simulink model "Template_v5_0_0_2026a_Original"  (R2026a)
settings: Solver=ode4  StopTime=tsim  FixedStep=baseRate  RelTol=1e-6  AbsTol=1e-6
undefined symbols (not defined in the file or in its folder): baseRate, dataRate, DiscIntNeverNeededParam, F_thrusters_BLACK, F_thrusters_BLUE, F_thrusters_RED, home_states_BLACK, home_states_BLUE, home_states_RED, IBLACK, IBLUE, init_states_BLACK, init_states_BLUE, init_states_RED, IRED, K_BLACK, K_BLUE, K_RED, labConsoleIP, mBLACK, mBLUE, mRED, Phase0_End, Phase1_End, Phase2_End, Phase3_End, Phase3_SubPhase1_End, Phase3_SubPhase2_End, Phase3_SubPhase3_End, Phase3_SubPhase4_End, Phase4_End, Phase5_End, platformSelection, PWMFreq, serverRate, simMode, tableDamping_BLACK, tableDamping_BLUE, tableDamping_RED, tableSlope, thrust_decay_BLACK, thrust_decay_BLUE, thrust_decay_RED, thruster_dist2CG_BLACK, thruster_dist2CG_BLUE, thruster_dist2CG_RED, xLength, yLength
libraries: simulink x18, dspinverses x3, nvidiaCommlib x1
(part 3 of 7)

== system Template_v5_0_0_2026a_Original/4 - Control/Disable Control (ARM) ==
  Action Port : ActionPort  ActionPortLabel=else
  Constant7 : Constant  Value=0
  Data Store Write12 : DataStoreWrite  DataStoreName=ARM_Control_Mode  IndexOptions=Index vector (dialog)  Indices=1  OutputSizes=1
  Mux : Mux  Inputs=3
  Zero : Constant  Value=0  OutDataTypeStr=Inherit: Inherit via back propagation
  Out1 : Outport
  wires:
  Mux/1 -> Out1/1
  Zero/1 -> Mux/3, Mux/1, Mux/2
  Constant7/1 -> Data Store Write12/1

== system Template_v5_0_0_2026a_Original/4 - Control/Disable Thrusters (BLACK) ==
  Action Port : ActionPort  ActionPortLabel=else
  Mux : Mux  Inputs=3
  Zero : Constant  Value=0  OutDataTypeStr=Inherit: Inherit via back propagation
  Out1 : Outport
  wires:
  Zero/1 -> Mux/3, Mux/1, Mux/2
  Mux/1 -> Out1/1

== system Template_v5_0_0_2026a_Original/4 - Control/Disable Thrusters (BLUE) ==
  Action Port : ActionPort  ActionPortLabel=else
  Mux : Mux  Inputs=3
  Zero : Constant  Value=0  OutDataTypeStr=Inherit: Inherit via back propagation
  Out1 : Outport
  wires:
  Zero/1 -> Mux/3, Mux/1, Mux/2
  Mux/1 -> Out1/1

== system Template_v5_0_0_2026a_Original/4 - Control/Disable Thrusters (RED) ==
  Action Port : ActionPort  ActionPortLabel=else
  Mux : Mux  Inputs=3
  Zero : Constant  Value=0  OutDataTypeStr=Inherit: Inherit via back propagation
  u : Outport
  wires:
  Zero/1 -> Mux/3, Mux/1, Mux/2
  Mux/1 -> u/1

== system Template_v5_0_0_2026a_Original/Check Connection/Change BLACK Behavior ==
  Action Port : ActionPort  ActionPortLabel=if(u1 == 2 & u2 == 0)
  Constant1 : Constant  OutDataTypeStr=int32
  UDP Send : MATLAB Function  TreatAsAtomicUnit=on
  wires:
  Constant1/1 -> UDP Send/1(data)

== system Template_v5_0_0_2026a_Original/Check Connection/Change BLUE Behavior ==
  Action Port : ActionPort  ActionPortLabel=if(u1 == 3 & u2 == 0)
  Constant1 : Constant  OutDataTypeStr=int32
  UDP Send : MATLAB Function  TreatAsAtomicUnit=on
  wires:
  Constant1/1 -> UDP Send/1(data)

== system Template_v5_0_0_2026a_Original/Check Connection/Change RED Behavior ==
  Action Port : ActionPort  ActionPortLabel=if(u1 == 1 & u2 == 0)
  Constant1 : Constant  OutDataTypeStr=int32
  UDP Send : MATLAB Function  TreatAsAtomicUnit=on
  wires:
  Constant1/1 -> UDP Send/1(data)

== system Template_v5_0_0_2026a_Original/Data Logger Subsystem/Data Logger ==
  Data : Inport
  MATLAB Function : MATLAB Function  TreatAsAtomicUnit=on
  MATLAB System : MATLABSystem  System=spot.hardware.CustomDataLogger
      mask Type: spot.hardware.CustomDataLogger
  wires:
  MATLAB Function/1(inputSize) -> MATLAB System/2
  Data/1 -> MATLAB System/1, MATLAB Function/1(Input)

== system Template_v5_0_0_2026a_Original/Live Data Streams/Live Stream 1 ==
  u : Inport
  Stream : MATLAB Function  TreatAsAtomicUnit=on
  Univ_Time : DataStoreRead  DataStoreName=Univ_Time  IndexOptions=Index vector (dialog)  Indices=1  OutputSizes=1
  WhoAmI : DataStoreRead  DataStoreName=WhoAmI  IndexOptions=Index vector (dialog)  Indices=1  OutputSizes=1
  isSim : DataStoreRead  DataStoreName=isSim  IndexOptions=Index vector (dialog)  Indices=1  OutputSizes=1
  wires:
  u/1 -> Stream/1(u)
  Univ_Time/1 -> Stream/2(t)
  WhoAmI/1 -> Stream/3(whoAmI)
  isSim/1 -> Stream/4(isSim)

== system Template_v5_0_0_2026a_Original/Live Data Streams/Live Stream 2 ==
  u : Inport
  Stream : MATLAB Function  TreatAsAtomicUnit=on
  Univ_Time : DataStoreRead  DataStoreName=Univ_Time  IndexOptions=Index vector (dialog)  Indices=1  OutputSizes=1
  WhoAmI : DataStoreRead  DataStoreName=WhoAmI  IndexOptions=Index vector (dialog)  Indices=1  OutputSizes=1
  isSim : DataStoreRead  DataStoreName=isSim  IndexOptions=Index vector (dialog)  Indices=1  OutputSizes=1
  wires:
  u/1 -> Stream/1(u)
  Univ_Time/1 -> Stream/2(t)
  WhoAmI/1 -> Stream/3(whoAmI)
  isSim/1 -> Stream/4(isSim)

== system Template_v5_0_0_2026a_Original/Live Data Streams/Live Stream 3 ==
  u : Inport
  Stream : MATLAB Function  TreatAsAtomicUnit=on
  Univ_Time : DataStoreRead  DataStoreName=Univ_Time  IndexOptions=Index vector (dialog)  Indices=1  OutputSizes=1
  WhoAmI : DataStoreRead  DataStoreName=WhoAmI  IndexOptions=Index vector (dialog)  Indices=1  OutputSizes=1
  isSim : DataStoreRead  DataStoreName=isSim  IndexOptions=Index vector (dialog)  Indices=1  OutputSizes=1
  wires:
  u/1 -> Stream/1(u)
  Univ_Time/1 -> Stream/2(t)
  WhoAmI/1 -> Stream/3(whoAmI)
  isSim/1 -> Stream/4(isSim)

== system Template_v5_0_0_2026a_Original/Live Data Streams/Live Stream 4 ==
  u : Inport
  Stream : MATLAB Function  TreatAsAtomicUnit=on
  Univ_Time : DataStoreRead  DataStoreName=Univ_Time  IndexOptions=Index vector (dialog)  Indices=1  OutputSizes=1
  WhoAmI : DataStoreRead  DataStoreName=WhoAmI  IndexOptions=Index vector (dialog)  Indices=1  OutputSizes=1
  isSim : DataStoreRead  DataStoreName=isSim  IndexOptions=Index vector (dialog)  Indices=1  OutputSizes=1
  wires:
  u/1 -> Stream/1(u)
  Univ_Time/1 -> Stream/2(t)
  WhoAmI/1 -> Stream/3(whoAmI)
  isSim/1 -> Stream/4(isSim)

== system Template_v5_0_0_2026a_Original/PhaseSpace Camera Code/Initialize Universal Time (Simulation) ==
  Action Port : ActionPort  ActionPortLabel=elseif(u1 == 1)
  Set Universal Time (If this is a simulation) : Clock
  Universal_Time : DataStoreWrite  DataStoreName=Univ_Time  IndexOptions=Index vector (dialog)  Indices=1  OutputSizes=1
  wires:
  Set Universal Time (If this is a simulation)/1 -> Universal_Time/1

== system Template_v5_0_0_2026a_Original/PhaseSpace Camera Code/Use Hardware to Obtain States ==
  Action Port : ActionPort  ActionPortLabel=if(u1 == 0)
  Demux : Demux  Outputs=[4,3,3,9]
  Demux1 : Demux  Outputs=[3,3,3]
  Receive and Process Phasespace Data : Subsystem
  Store BLACK Data : Subsystem
  Store BLUE Data : Subsystem
  Store RED Data : Subsystem
  wires:
  Receive and Process Phasespace Data/1(PhaseSpace Data) -> Demux/1
  Demux/1 -> Store RED Data/1(RED Data)
  Demux/2 -> Store BLACK Data/1(BLACK Data)
  Demux/3 -> Store BLUE Data/1(BLUE Data)
  Demux/4 -> Demux1/1
  Demux1/1 -> Store RED Data/2(RED Velocities)
  Demux1/2 -> Store BLACK Data/2(BLACK Velocities)
  Demux1/3 -> Store BLUE Data/2(BLUE Velocities)
  Receive and Process Phasespace Data/2(PhaseSpace Clock) -> Store RED Data/3(PS Clock), Store BLACK Data/3(PS Clock), Store BLUE Data/3(PS Clock)

== system Template_v5_0_0_2026a_Original/Platform Identification/Subsystem ==
  Action Port : ActionPort  ActionPortLabel=if(u1 == 0)
  Data Store Write : DataStoreWrite  DataStoreName=WhoAmI  IndexOptions=Index vector (dialog)  Indices=1  OutputSizes=1
  WhoAmI : MATLABSystem  System=spot.hardware.IdentifyPlatform  SampleTime=baseRate
      mask Type: spot.hardware.IdentifyPlatform
  wires:
  WhoAmI/1 -> Data Store Write/1

== system Template_v5_0_0_2026a_Original/Receive Data from Orin/Subsystem ==
  Action Port : ActionPort  ActionPortLabel=if(u1 == 0)
  Cast To Double{,1..3} (4 alike) : DataTypeConversion  OutDataTypeStr=double  SaturateOnIntegerOverflow=off  RndMeth=Floor
  Data Store Write : DataStoreWrite  DataStoreName=VIS_Measured_States  IndexOptions=Index vector (dialog)  Indices=1  OutputSizes=1
  Data Store Write1 : DataStoreWrite  DataStoreName=VIS_Confidence  IndexOptions=Index vector (dialog)  Indices=1  OutputSizes=1
  Demux : Demux
  Mux : Mux  Inputs=3
  Terminator : Terminator
  Terminator1 : Terminator
  UDP Receive : MATLAB Function  TreatAsAtomicUnit=on
  wires:
  Demux/1 -> Cast To Double/1
  Demux/2 -> Cast To Double1/1
  Demux/3 -> Cast To Double2/1
  Demux/4 -> Cast To Double3/1
  Cast To Double/1 -> Mux/1
  Cast To Double1/1 -> Mux/2
  Cast To Double2/1 -> Mux/3
  Mux/1 -> Data Store Write/1
  Cast To Double3/1 -> Data Store Write1/1
  UDP Receive/1(data) -> Demux/1
  UDP Receive/2(newPackets) -> Terminator/1
  UDP Receive/3(age) -> Terminator1/1

== system Template_v5_0_0_2026a_Original/Robotic Arm Code/Change ARM Behavior ==
  note: Reads the encoders here (priority 21, before the controllers); sends the PWM input (ARM_Controls, from Robotic Arm Code) at the end of the step. See help spot.hardware.ArmPWM.
  PWM : Inport
  Action Port : ActionPort  ActionPortLabel=if(u1 == 1 & u2 == 0)
  Data Store Write : DataStoreWrite  DataStoreName=ARM_Measured_States  IndexOptions=Index vector (dialog)  Indices=1  OutputSizes=1
  Data Store Write1 : DataStoreWrite  DataStoreName=ARM_Measured_PWM  IndexOptions=Index vector (dialog)  Indices=1  OutputSizes=1
  Data Store Write2 : DataStoreWrite  DataStoreName=ARM_Servo_Status  IndexOptions=Index vector (dialog)  Indices=1  OutputSizes=1
  Dynamixel Arm (PWM) : MATLABSystem  System=spot.hardware.ArmPWM  Port=/dev/ttyUSB0  PWMLimit=885  ZeroReturnDelay=off  MinPosition=1024  MaxPosition=3072
      mask Type: spot.hardware.ArmPWM
  Mux : Mux  Inputs=2
  wires:
  Dynamixel Arm (PWM)/1 -> Mux/1
  Dynamixel Arm (PWM)/2 -> Mux/2
  Mux/1 -> Data Store Write/1
  Dynamixel Arm (PWM)/3 -> Data Store Write1/1
  Dynamixel Arm (PWM)/4 -> Data Store Write2/1
  PWM/1 -> Dynamixel Arm (PWM)/1

== system Template_v5_0_0_2026a_Original/Send Data to Orin/Subsystem ==
  Action Port : ActionPort  ActionPortLabel=if(u1 == 0)
  BLACK States : DataStoreRead  DataStoreName=BLACK_Measured_States  IndexOptions=Index vector (dialog)  Indices=1  OutputSizes=1
  BLUE States : DataStoreRead  DataStoreName=BLUE_Measured_States  IndexOptions=Index vector (dialog)  Indices=1  OutputSizes=1
  Mux : Mux
  RED States : DataStoreRead  DataStoreName=RED_Measured_States  IndexOptions=Index vector (dialog)  Indices=1  OutputSizes=1
  Time : DataStoreRead  DataStoreName=Univ_Time  IndexOptions=Index vector (dialog)  Indices=1  OutputSizes=1
  UDP Send : MATLAB Function  TreatAsAtomicUnit=on
  wires:
  Time/1 -> Mux/1
  RED States/1 -> Mux/2
  BLACK States/1 -> Mux/3
  BLUE States/1 -> Mux/4
  Mux/1 -> UDP Send/1(data)

== system Template_v5_0_0_2026a_Original/Simulate Plant Dynamics/BLACK Dynamics ==
  Add Noise : RandomNumber  Variance=1e-9  SampleTime=baseRate
  Calculated & Store Measured States : Subsystem
  Calculated & Store True States : Subsystem
  Data @ Measurement Rate : Subsystem
  Dynamics Model for BLACK : Subsystem  SystemSampleTime=serverRate
      settings: PortSchema="{\"entries\":[{\"content\":{\"sides\":[{\"content\":{\"connectorIds\":[\"In1\"]},\"type\":\"ConnectorPlacement.EquallySpacedRectSide\",\"uuid\":\"9df3cfb7-f920-4c45-b004-2d63eab5f007\"},{\"content\":{\"side\":\"RIGHT\"},\"type\":\"ConnectorPlacement.EquallySpacedRectSide\",\"uuid\":\"24f4b70f-864f-4cab-bc2b-b450467a01b3\"},{\"content\":{\"connectorIds\":[\"Out1\"],\"side\":\"TOP\"},\"type\":\"ConnectorPlacement.EquallySpacedRectSide\",\"uuid\":\"64c0236c-f70a-4099-950e-ee3e8643e7f2\"}]},\"type\":\"ConnectorPlacement.EquallySpacedConnector\",\"uuid\":\"dd7c693a-185b-4c5f-873e-b9df56bea395\"}],\"packageUris\":[\"http://schema.mathworks.com/mf0/Connector/R2020b\"],\"version\":\"1.0\"}"
  Saturated Control Commands for BLACK : DataStoreRead  DataStoreName=BLACK_Saturated_Controls  IndexOptions=Index vector (dialog)  Indices=1  OutputSizes=1
  Sum : Sum  Inputs=++|
  wires:
  Dynamics Model for BLACK/1(states) -> Sum/2, Calculated & Store True States/1(y)
  Data @ Measurement Rate/2(Time Step) -> Calculated & Store Measured States/2(dt)
  Saturated Control Commands for BLACK/1 -> Dynamics Model for BLACK/1(control_inputs)
  Data @ Measurement Rate/1(Data Held) -> Calculated & Store Measured States/1(y)
  Sum/1 -> Data @ Measurement Rate/1(Data Input)
  Add Noise/1 -> Sum/1

== system Template_v5_0_0_2026a_Original/Simulate Plant Dynamics/BLUE Dynamics ==
  Add Noise : RandomNumber  Variance=1e-9  SampleTime=baseRate
  BLUE  Dynamics Model : Subsystem  SystemSampleTime=serverRate
      settings: PortSchema="{\"entries\":[{\"content\":{\"sides\":[{\"content\":{\"connectorIds\":[\"In1\"]},\"type\":\"ConnectorPlacement.EquallySpacedRectSide\",\"uuid\":\"9df3cfb7-f920-4c45-b004-2d63eab5f007\"},{\"content\":{\"side\":\"RIGHT\"},\"type\":\"ConnectorPlacement.EquallySpacedRectSide\",\"uuid\":\"24f4b70f-864f-4cab-bc2b-b450467a01b3\"},{\"content\":{\"connectorIds\":[\"Out1\"],\"side\":\"TOP\"},\"type\":\"ConnectorPlacement.EquallySpacedRectSide\",\"uuid\":\"64c0236c-f70a-4099-950e-ee3e8643e7f2\"}]},\"type\":\"ConnectorPlacement.EquallySpacedConnector\",\"uuid\":\"dd7c693a-185b-4c5f-873e-b9df56bea395\"}],\"packageUris\":[\"http://schema.mathworks.com/mf0/Connector/R2020b\"],\"version\":\"1.0\"}"
  Calculated & Store Measured States : Subsystem
  Calculated & Store True States : Subsystem
  Data @ Measurement Rate : Subsystem
  Saturated Control Commands for BLUE : DataStoreRead  DataStoreName=BLUE_Saturated_Controls  IndexOptions=Index vector (dialog)  Indices=1  OutputSizes=1
  Sum1 : Sum  Inputs=++|
  wires:
  Saturated Control Commands for BLUE/1 -> BLUE  Dynamics Model/1(control_inputs)
  Data @ Measurement Rate/2(Time Step) -> Calculated & Store Measured States/2(dt)
  Add Noise/1 -> Sum1/1
  BLUE  Dynamics Model/1(states) -> Sum1/2, Calculated & Store True States/1(y)
  Sum1/1 -> Data @ Measurement Rate/1(Data Input)
  Data @ Measurement Rate/1(Data Held) -> Calculated & Store Measured States/1(y)

== system Template_v5_0_0_2026a_Original/Simulate Plant Dynamics/RED and ARM Dynamics ==
  Constant : Constant  Value=platformSelection
  If : If  IfExpression=u1 == 4 | u1 == 5 | u1 == 10 | u1 == 11
  RED + ARM : Subsystem  TreatAsAtomicUnit=on
  RED Only : Subsystem  TreatAsAtomicUnit=on
  wires:
  If/1 -> RED + ARM/Action
  Constant/1 -> If/1
  If/2 -> RED Only/Action

== system Template_v5_0_0_2026a_Original/Thruster & Float Control Code/Change BLACK Behavior ==
  note: Calculate the percentage of time each thruster must be on, and send to the PWM blocks.
  note: Using the attitude, rotate the forces into the body frame.
  note: Calculate which thrusters must be turned on and for how long.
  Action Port : ActionPort  ActionPortLabel=if(u1 == 2 | u2 == 1)
  BLACK Controls : DataStoreRead  DataStoreName=BLACK_Controls  IndexOptions=Index vector (dialog)  Indices=1  OutputSizes=1
  BLACK States : DataStoreRead  DataStoreName=BLACK_Measured_States  IndexOptions=Index vector (dialog)  Indices=1  OutputSizes=1
  Calculate Duty Cycle : Subsystem
  Data Store Write2 : DataStoreWrite  DataStoreName=BLACK_Saturated_Controls  IndexOptions=Index vector (dialog)  Indices=1  OutputSizes=1
  Demux1 : Demux  Outputs=[2,1]
  Demux2 : Demux  Outputs=[2,1,6]
  Mux : Mux  Inputs=2
  Rotate Forces to Body : Subsystem
  Terminator : Terminator
  Terminator1 : Terminator
  BLACK DC : Outport  VectorParamsAs1DForOutWhenUnconnected=off
  wires:
  Calculate Duty Cycle/2(Saturated Forces Moments) -> Data Store Write2/1
  Rotate Forces to Body/1(F_b) -> Mux/1
  Demux1/2 -> Mux/2
  Calculate Duty Cycle/1(Duty Cycle) -> BLACK DC/1
  Mux/1 -> Calculate Duty Cycle/1("[Fx_b; Fy_b; Tz]")
  BLACK Controls/1 -> Demux1/1
  Demux1/1 -> Rotate Forces to Body/1("F_I ")
  BLACK States/1 -> Demux2/1
  Demux2/1 -> Terminator/1
  Demux2/3 -> Terminator1/1
  Demux2/2 -> Calculate Duty Cycle/2(Measured Attitude), Rotate Forces to Body/2(Rz)

== system Template_v5_0_0_2026a_Original/Thruster & Float Control Code/Change BLUE Behavior ==
  note: Calculate the percentage of time each thruster must be on, and send to the PWM blocks.
  note: Using the attitude, rotate the forces into the body frame.
  note: Calculate which thrusters must be turned on and for how long.
  Action Port : ActionPort  ActionPortLabel=if(u1 == 3 | u2 == 1)
  Calculate Duty Cycle : Subsystem
  Data Store Read : DataStoreRead  DataStoreName=BLUE_Controls  IndexOptions=Index vector (dialog)  Indices=1  OutputSizes=1
  Data Store Read1 : DataStoreRead  DataStoreName=BLUE_Measured_States  IndexOptions=Index vector (dialog)  Indices=1  OutputSizes=1
  Data Store Write3 : DataStoreWrite  DataStoreName=BLUE_Saturated_Controls  IndexOptions=Index vector (dialog)  Indices=1  OutputSizes=1
  Demux : Demux  Outputs=[2,1]
  Demux1 : Demux  Outputs=[2,1,6]
  Mux1 : Mux  Inputs=2
  Rotate Forces to Body : Subsystem
  Terminator : Terminator
  Terminator1 : Terminator
  BLUE DC : Outport  VectorParamsAs1DForOutWhenUnconnected=off
  wires:
  Calculate Duty Cycle/1(Duty Cycle) -> BLUE DC/1
  Rotate Forces to Body/1(F_b) -> Mux1/1
  Demux/2 -> Mux1/2
  Mux1/1 -> Calculate Duty Cycle/1("[Fx_b; Fy_b; Tz]")
  Calculate Duty Cycle/2(Saturated Forces Moments) -> Data Store Write3/1
  Data Store Read/1 -> Demux/1
  Demux/1 -> Rotate Forces to Body/1("F_I ")
  Data Store Read1/1 -> Demux1/1
  Demux1/2 -> Calculate Duty Cycle/2(Measured Attitude), Rotate Forces to Body/2(Rz)
  Demux1/1 -> Terminator/1
  Demux1/3 -> Terminator1/1

== system Template_v5_0_0_2026a_Original/Thruster & Float Control Code/Change RED Behavior ==
  note: Calculate which thrusters must be turned on and for how long.
  note: Calculate the percentage of time each thruster must be on, and send to the PWM blocks.
  note: Using the attitude, rotate the forces into the body frame.
  Action Port : ActionPort  ActionPortLabel=if(u1 == 1 | u2 == 1)
  Calculate Duty Cycle : Subsystem
  Data Store Read : DataStoreRead  DataStoreName=RED_Controls  IndexOptions=Index vector (dialog)  Indices=1  OutputSizes=1
  Data Store Read1 : DataStoreRead  DataStoreName=RED_Measured_States  IndexOptions=Index vector (dialog)  Indices=1  OutputSizes=1
  Data Store Write1 : DataStoreWrite  DataStoreName=RED_Saturated_Controls  IndexOptions=Index vector (dialog)  Indices=1  OutputSizes=1
  Demux : Demux  Outputs=[2,1]
  Demux1 : Demux  Outputs=[2,1,6]
  Mux1 : Mux  Inputs=2
  Rotate Forces to Body : Subsystem
  Terminator : Terminator
  Terminator1 : Terminator
  RED DC : Outport  VectorParamsAs1DForOutWhenUnconnected=off
  wires:
  Demux/1 -> Rotate Forces to Body/1("F_I ")
  Mux1/1 -> Calculate Duty Cycle/1("[Fx_b; Fy_b; Tz]")
  Demux/2 -> Mux1/2
  Demux1/2 -> Calculate Duty Cycle/2(Measured Attitude), Rotate Forces to Body/2(Rz)
  Rotate Forces to Body/1(F_b) -> Mux1/1
  Data Store Read/1 -> Demux/1
  Demux1/1 -> Terminator/1
  Demux1/3 -> Terminator1/1
  Data Store Read1/1 -> Demux1/1
  Calculate Duty Cycle/2(Saturated Forces Moments) -> Data Store Write1/1
  Calculate Duty Cycle/1(Duty Cycle) -> RED DC/1

== system Template_v5_0_0_2026a_Original/1 - Experiment Logic/Phase #2: Initial Position/Desired Joint Angles RED ==
  Constant1 : Constant  Value=pi/2
  Constant2 : Constant  Value=0
  Constant3 : Constant  Value=pi/2
  Mux : Mux  Inputs=3
  Target Array : Outport
  wires:
  Mux/1 -> Target Array/1
  Constant3/1 -> Mux/1
  Constant1/1 -> Mux/2
  Constant2/1 -> Mux/3

== system Template_v5_0_0_2026a_Original/1 - Experiment Logic/Phase #2: Initial Position/Desired Position BLACK ==
  Desired States (BLACK) : Constant  Value=init_states_BLACK  SampleTime=-1
  Target Array : Outport
  wires:
  Desired States (BLACK)/1 -> Target Array/1

== system Template_v5_0_0_2026a_Original/1 - Experiment Logic/Phase #2: Initial Position/Desired Position BLUE ==
  Desired States (BLUE) : Constant  Value=init_states_BLUE  SampleTime=-1
  Target Array : Outport
  wires:
  Desired States (BLUE)/1 -> Target Array/1

== system Template_v5_0_0_2026a_Original/1 - Experiment Logic/Phase #2: Initial Position/Desired Position RED ==
  Constant2 : Constant  Value=init_states_RED
  Target Array : Outport
  wires:
  Constant2/1 -> Target Array/1

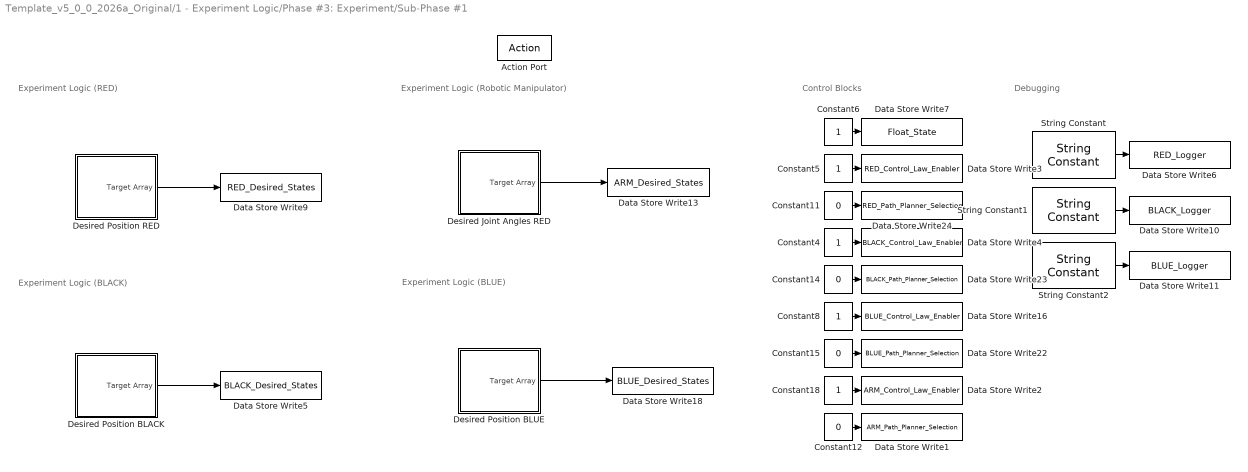
== system Template_v5_0_0_2026a_Original/1 - Experiment Logic/Phase #3: Experiment/Sub-Phase #1 ==
  note: Experiment Logic (BLUE)
  note: Experiment Logic (Robotic Manipulator)
  note: Experiment Logic (RED)
  note: Experiment Logic (BLACK)
  note: Control Blocks
  note: Debugging
  Action Port : ActionPort  ActionPortLabel=if(u1 < u2)
  Constant{11..12,14..15} (4 alike) : Constant  Value=0
  Constant{4..6,8,18} (5 alike) : Constant
  Data Store Write1 : DataStoreWrite  DataStoreName=ARM_Path_Planner_Selection  IndexOptions=Index vector (dialog)  Indices=1  OutputSizes=1
  Data Store Write10 : DataStoreWrite  DataStoreName=BLACK_Logger  IndexOptions=Index vector (dialog)  Indices=1  OutputSizes=1
  Data Store Write11 : DataStoreWrite  DataStoreName=BLUE_Logger  IndexOptions=Index vector (dialog)  Indices=1  OutputSizes=1
  Data Store Write13 : DataStoreWrite  DataStoreName=ARM_Desired_States  IndexOptions=Index vector (dialog)  Indices=1  OutputSizes=1
  Data Store Write16 : DataStoreWrite  DataStoreName=BLUE_Control_Law_Enabler  IndexOptions=Index vector (dialog)  Indices=1  OutputSizes=1
  Data Store Write18 : DataStoreWrite  DataStoreName=BLUE_Desired_States  IndexOptions=Index vector (dialog)  Indices=1  OutputSizes=1
  Data Store Write2 : DataStoreWrite  DataStoreName=ARM_Control_Law_Enabler  IndexOptions=Index vector (dialog)  Indices=1  OutputSizes=1
  Data Store Write22 : DataStoreWrite  DataStoreName=BLUE_Path_Planner_Selection  IndexOptions=Index vector (dialog)  Indices=1  OutputSizes=1
  Data Store Write23 : DataStoreWrite  DataStoreName=BLACK_Path_Planner_Selection  IndexOptions=Index vector (dialog)  Indices=1  OutputSizes=1
  Data Store Write24 : DataStoreWrite  DataStoreName=RED_Path_Planner_Selection  IndexOptions=Index vector (dialog)  Indices=1  OutputSizes=1
  Data Store Write3 : DataStoreWrite  DataStoreName=RED_Control_Law_Enabler  IndexOptions=Index vector (dialog)  Indices=1  OutputSizes=1
  Data Store Write4 : DataStoreWrite  DataStoreName=BLACK_Control_Law_Enabler  IndexOptions=Index vector (dialog)  Indices=1  OutputSizes=1
  Data Store Write5 : DataStoreWrite  DataStoreName=BLACK_Desired_States  IndexOptions=Index vector (dialog)  Indices=1  OutputSizes=1
  Data Store Write6 : DataStoreWrite  DataStoreName=RED_Logger  IndexOptions=Index vector (dialog)  Indices=1  OutputSizes=1
  Data Store Write7 : DataStoreWrite  DataStoreName=Float_State  IndexOptions=Index vector (dialog)  Indices=1  OutputSizes=1
  Data Store Write9 : DataStoreWrite  DataStoreName=RED_Desired_States  IndexOptions=Index vector (dialog)  Indices=1  OutputSizes=1
  Desired Joint Angles RED : Subsystem
  Desired Position BLACK : Subsystem
  Desired Position BLUE : Subsystem
  Desired Position RED : Subsystem
  String Constant : StringConstant  String="\"Chaser: Running Phase 3 Sub-Phase 1\""
  String Constant1 : StringConstant  String="\"Target: Running Phase 3 Sub-Phase 1\""
  String Constant2 : StringConstant  String="\"Obstacle: Running Phase 3 Sub-Phase 1\""
  wires:
  Desired Position BLUE/1(Target Array) -> Data Store Write18/1
  Desired Position RED/1(Target Array) -> Data Store Write9/1
  Desired Joint Angles RED/1(Target Array) -> Data Store Write13/1
  Constant12/1 -> Data Store Write1/1
  Constant18/1 -> Data Store Write2/1
  Constant6/1 -> Data Store Write7/1
  Constant15/1 -> Data Store Write22/1
  Constant14/1 -> Data Store Write23/1
  Constant5/1 -> Data Store Write3/1
  Constant11/1 -> Data Store Write24/1
  Constant8/1 -> Data Store Write16/1
  Constant4/1 -> Data Store Write4/1
  String Constant2/1 -> Data Store Write11/1
  String Constant1/1 -> Data Store Write10/1
  String Constant/1 -> Data Store Write6/1
  Desired Position BLACK/1(Target Array) -> Data Store Write5/1

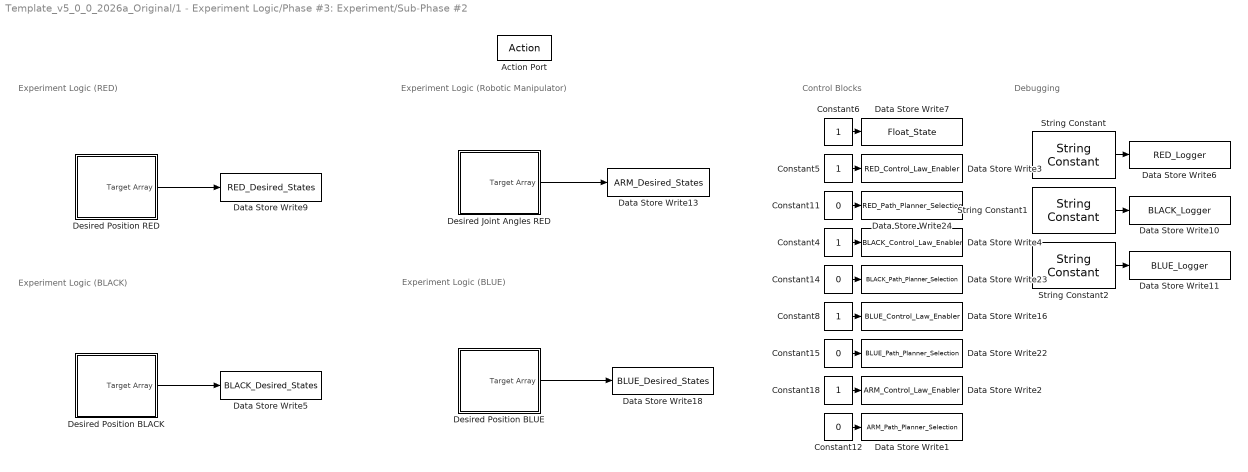
== system Template_v5_0_0_2026a_Original/1 - Experiment Logic/Phase #3: Experiment/Sub-Phase #2 ==
  note: Experiment Logic (BLUE)
  note: Experiment Logic (Robotic Manipulator)
  note: Experiment Logic (RED)
  note: Experiment Logic (BLACK)
  note: Control Blocks
  note: Debugging
  Action Port : ActionPort  ActionPortLabel=elseif((u1 < u3 & u1 >= u2))
  Constant{11..12,14..15} (4 alike) : Constant  Value=0
  Constant{4..6,8,18} (5 alike) : Constant
  Data Store Write1 : DataStoreWrite  DataStoreName=ARM_Path_Planner_Selection  IndexOptions=Index vector (dialog)  Indices=1  OutputSizes=1
  Data Store Write10 : DataStoreWrite  DataStoreName=BLACK_Logger  IndexOptions=Index vector (dialog)  Indices=1  OutputSizes=1
  Data Store Write11 : DataStoreWrite  DataStoreName=BLUE_Logger  IndexOptions=Index vector (dialog)  Indices=1  OutputSizes=1
  Data Store Write13 : DataStoreWrite  DataStoreName=ARM_Desired_States  IndexOptions=Index vector (dialog)  Indices=1  OutputSizes=1
  Data Store Write16 : DataStoreWrite  DataStoreName=BLUE_Control_Law_Enabler  IndexOptions=Index vector (dialog)  Indices=1  OutputSizes=1
  Data Store Write18 : DataStoreWrite  DataStoreName=BLUE_Desired_States  IndexOptions=Index vector (dialog)  Indices=1  OutputSizes=1
  Data Store Write2 : DataStoreWrite  DataStoreName=ARM_Control_Law_Enabler  IndexOptions=Index vector (dialog)  Indices=1  OutputSizes=1
  Data Store Write22 : DataStoreWrite  DataStoreName=BLUE_Path_Planner_Selection  IndexOptions=Index vector (dialog)  Indices=1  OutputSizes=1
  Data Store Write23 : DataStoreWrite  DataStoreName=BLACK_Path_Planner_Selection  IndexOptions=Index vector (dialog)  Indices=1  OutputSizes=1
  Data Store Write24 : DataStoreWrite  DataStoreName=RED_Path_Planner_Selection  IndexOptions=Index vector (dialog)  Indices=1  OutputSizes=1
  Data Store Write3 : DataStoreWrite  DataStoreName=RED_Control_Law_Enabler  IndexOptions=Index vector (dialog)  Indices=1  OutputSizes=1
  Data Store Write4 : DataStoreWrite  DataStoreName=BLACK_Control_Law_Enabler  IndexOptions=Index vector (dialog)  Indices=1  OutputSizes=1
  Data Store Write5 : DataStoreWrite  DataStoreName=BLACK_Desired_States  IndexOptions=Index vector (dialog)  Indices=1  OutputSizes=1
  Data Store Write6 : DataStoreWrite  DataStoreName=RED_Logger  IndexOptions=Index vector (dialog)  Indices=1  OutputSizes=1
  Data Store Write7 : DataStoreWrite  DataStoreName=Float_State  IndexOptions=Index vector (dialog)  Indices=1  OutputSizes=1
  Data Store Write9 : DataStoreWrite  DataStoreName=RED_Desired_States  IndexOptions=Index vector (dialog)  Indices=1  OutputSizes=1
  Desired Joint Angles RED : Subsystem
  Desired Position BLACK : Subsystem
  Desired Position BLUE : Subsystem
  Desired Position RED : Subsystem
  String Constant : StringConstant  String="\"Chaser: Running Phase 3 Sub-Phase 2\""
  String Constant1 : StringConstant  String="\"Target: Running Phase 3 Sub-Phase 2\""
  String Constant2 : StringConstant  String="\"Obstacle: Running Phase 3 Sub-Phase 2\""
  wires:
  Desired Position BLUE/1(Target Array) -> Data Store Write18/1
  Desired Position RED/1(Target Array) -> Data Store Write9/1
  Desired Joint Angles RED/1(Target Array) -> Data Store Write13/1
  Constant12/1 -> Data Store Write1/1
  Constant18/1 -> Data Store Write2/1
  Constant6/1 -> Data Store Write7/1
  Constant15/1 -> Data Store Write22/1
  Constant14/1 -> Data Store Write23/1
  Constant5/1 -> Data Store Write3/1
  Constant11/1 -> Data Store Write24/1
  Constant8/1 -> Data Store Write16/1
  Constant4/1 -> Data Store Write4/1
  String Constant2/1 -> Data Store Write11/1
  String Constant1/1 -> Data Store Write10/1
  String Constant/1 -> Data Store Write6/1
  Desired Position BLACK/1(Target Array) -> Data Store Write5/1

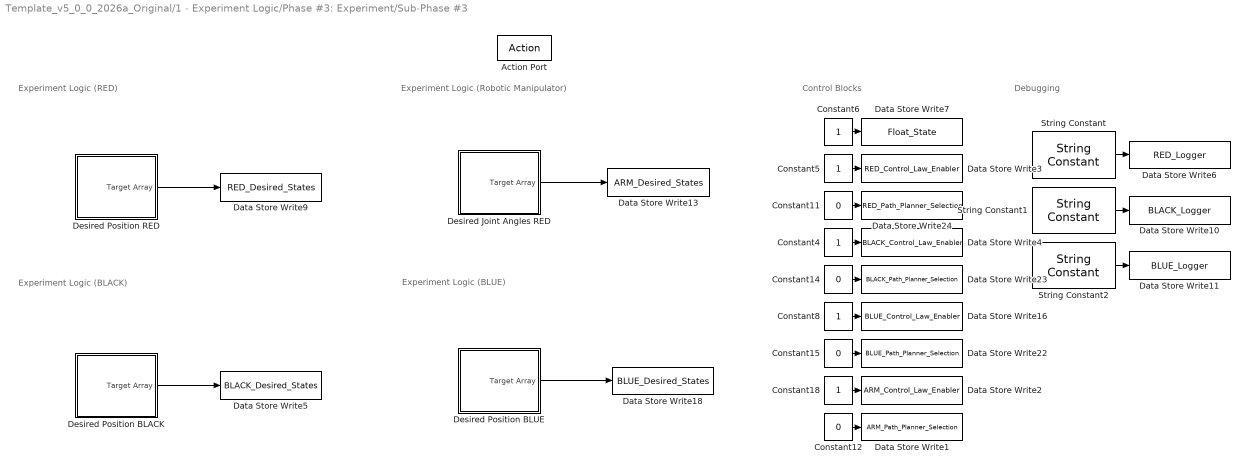
== system Template_v5_0_0_2026a_Original/1 - Experiment Logic/Phase #3: Experiment/Sub-Phase #3 ==
  note: Experiment Logic (BLUE)
  note: Experiment Logic (Robotic Manipulator)
  note: Experiment Logic (RED)
  note: Experiment Logic (BLACK)
  note: Control Blocks
  note: Debugging
  Action Port : ActionPort  ActionPortLabel=elseif((u1 < u4 & u1 >= u3))
  Constant{11..12,14..15} (4 alike) : Constant  Value=0
  Constant{4..6,8,18} (5 alike) : Constant
  Data Store Write1 : DataStoreWrite  DataStoreName=ARM_Path_Planner_Selection  IndexOptions=Index vector (dialog)  Indices=1  OutputSizes=1
  Data Store Write10 : DataStoreWrite  DataStoreName=BLACK_Logger  IndexOptions=Index vector (dialog)  Indices=1  OutputSizes=1
  Data Store Write11 : DataStoreWrite  DataStoreName=BLUE_Logger  IndexOptions=Index vector (dialog)  Indices=1  OutputSizes=1
  Data Store Write13 : DataStoreWrite  DataStoreName=ARM_Desired_States  IndexOptions=Index vector (dialog)  Indices=1  OutputSizes=1
  Data Store Write16 : DataStoreWrite  DataStoreName=BLUE_Control_Law_Enabler  IndexOptions=Index vector (dialog)  Indices=1  OutputSizes=1
  Data Store Write18 : DataStoreWrite  DataStoreName=BLUE_Desired_States  IndexOptions=Index vector (dialog)  Indices=1  OutputSizes=1
  Data Store Write2 : DataStoreWrite  DataStoreName=ARM_Control_Law_Enabler  IndexOptions=Index vector (dialog)  Indices=1  OutputSizes=1
  Data Store Write22 : DataStoreWrite  DataStoreName=BLUE_Path_Planner_Selection  IndexOptions=Index vector (dialog)  Indices=1  OutputSizes=1
  Data Store Write23 : DataStoreWrite  DataStoreName=BLACK_Path_Planner_Selection  IndexOptions=Index vector (dialog)  Indices=1  OutputSizes=1
  Data Store Write24 : DataStoreWrite  DataStoreName=RED_Path_Planner_Selection  IndexOptions=Index vector (dialog)  Indices=1  OutputSizes=1
  Data Store Write3 : DataStoreWrite  DataStoreName=RED_Control_Law_Enabler  IndexOptions=Index vector (dialog)  Indices=1  OutputSizes=1
  Data Store Write4 : DataStoreWrite  DataStoreName=BLACK_Control_Law_Enabler  IndexOptions=Index vector (dialog)  Indices=1  OutputSizes=1
  Data Store Write5 : DataStoreWrite  DataStoreName=BLACK_Desired_States  IndexOptions=Index vector (dialog)  Indices=1  OutputSizes=1
  Data Store Write6 : DataStoreWrite  DataStoreName=RED_Logger  IndexOptions=Index vector (dialog)  Indices=1  OutputSizes=1
  Data Store Write7 : DataStoreWrite  DataStoreName=Float_State  IndexOptions=Index vector (dialog)  Indices=1  OutputSizes=1
  Data Store Write9 : DataStoreWrite  DataStoreName=RED_Desired_States  IndexOptions=Index vector (dialog)  Indices=1  OutputSizes=1
  Desired Joint Angles RED : Subsystem
  Desired Position BLACK : Subsystem
  Desired Position BLUE : Subsystem
  Desired Position RED : Subsystem
  String Constant : StringConstant  String="\"Chaser: Running Phase 3 Sub-Phase 3\""
  String Constant1 : StringConstant  String="\"Target: Running Phase 3 Sub-Phase 3\""
  String Constant2 : StringConstant  String="\"Obstacle: Running Phase 3 Sub-Phase 3\""
  wires:
  Desired Position BLUE/1(Target Array) -> Data Store Write18/1
  Desired Position RED/1(Target Array) -> Data Store Write9/1
  Desired Joint Angles RED/1(Target Array) -> Data Store Write13/1
  Constant12/1 -> Data Store Write1/1
  Constant18/1 -> Data Store Write2/1
  Constant6/1 -> Data Store Write7/1
  Constant15/1 -> Data Store Write22/1
  Constant14/1 -> Data Store Write23/1
  Constant5/1 -> Data Store Write3/1
  Constant11/1 -> Data Store Write24/1
  Constant8/1 -> Data Store Write16/1
  Constant4/1 -> Data Store Write4/1
  String Constant2/1 -> Data Store Write11/1
  String Constant1/1 -> Data Store Write10/1
  String Constant/1 -> Data Store Write6/1
  Desired Position BLACK/1(Target Array) -> Data Store Write5/1

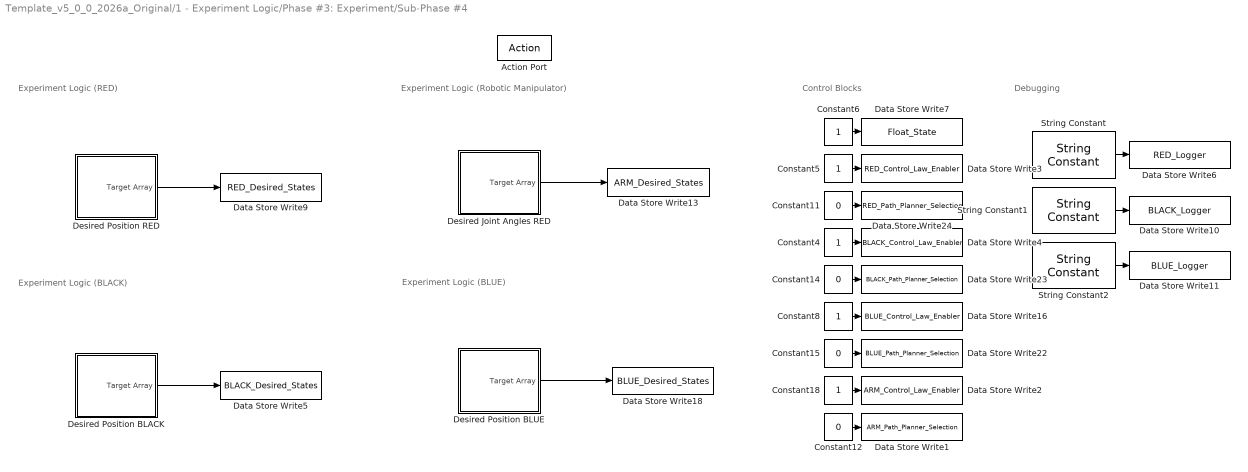
== system Template_v5_0_0_2026a_Original/1 - Experiment Logic/Phase #3: Experiment/Sub-Phase #4 ==
  note: Experiment Logic (BLUE)
  note: Experiment Logic (Robotic Manipulator)
  note: Experiment Logic (RED)
  note: Experiment Logic (BLACK)
  note: Control Blocks
  note: Debugging
  Action Port : ActionPort  ActionPortLabel=elseif( (u1 < u5 & u1 >= u4))
  Constant{11..12,14..15} (4 alike) : Constant  Value=0
  Constant{4..6,8,18} (5 alike) : Constant
  Data Store Write1 : DataStoreWrite  DataStoreName=ARM_Path_Planner_Selection  IndexOptions=Index vector (dialog)  Indices=1  OutputSizes=1
  Data Store Write10 : DataStoreWrite  DataStoreName=BLACK_Logger  IndexOptions=Index vector (dialog)  Indices=1  OutputSizes=1
  Data Store Write11 : DataStoreWrite  DataStoreName=BLUE_Logger  IndexOptions=Index vector (dialog)  Indices=1  OutputSizes=1
  Data Store Write13 : DataStoreWrite  DataStoreName=ARM_Desired_States  IndexOptions=Index vector (dialog)  Indices=1  OutputSizes=1
  Data Store Write16 : DataStoreWrite  DataStoreName=BLUE_Control_Law_Enabler  IndexOptions=Index vector (dialog)  Indices=1  OutputSizes=1
  Data Store Write18 : DataStoreWrite  DataStoreName=BLUE_Desired_States  IndexOptions=Index vector (dialog)  Indices=1  OutputSizes=1
  Data Store Write2 : DataStoreWrite  DataStoreName=ARM_Control_Law_Enabler  IndexOptions=Index vector (dialog)  Indices=1  OutputSizes=1
  Data Store Write22 : DataStoreWrite  DataStoreName=BLUE_Path_Planner_Selection  IndexOptions=Index vector (dialog)  Indices=1  OutputSizes=1
  Data Store Write23 : DataStoreWrite  DataStoreName=BLACK_Path_Planner_Selection  IndexOptions=Index vector (dialog)  Indices=1  OutputSizes=1
  Data Store Write24 : DataStoreWrite  DataStoreName=RED_Path_Planner_Selection  IndexOptions=Index vector (dialog)  Indices=1  OutputSizes=1
  Data Store Write3 : DataStoreWrite  DataStoreName=RED_Control_Law_Enabler  IndexOptions=Index vector (dialog)  Indices=1  OutputSizes=1
  Data Store Write4 : DataStoreWrite  DataStoreName=BLACK_Control_Law_Enabler  IndexOptions=Index vector (dialog)  Indices=1  OutputSizes=1
  Data Store Write5 : DataStoreWrite  DataStoreName=BLACK_Desired_States  IndexOptions=Index vector (dialog)  Indices=1  OutputSizes=1
  Data Store Write6 : DataStoreWrite  DataStoreName=RED_Logger  IndexOptions=Index vector (dialog)  Indices=1  OutputSizes=1
  Data Store Write7 : DataStoreWrite  DataStoreName=Float_State  IndexOptions=Index vector (dialog)  Indices=1  OutputSizes=1
  Data Store Write9 : DataStoreWrite  DataStoreName=RED_Desired_States  IndexOptions=Index vector (dialog)  Indices=1  OutputSizes=1
  Desired Joint Angles RED : Subsystem
  Desired Position BLACK : Subsystem
  Desired Position BLUE : Subsystem
  Desired Position RED : Subsystem
  String Constant : StringConstant  String="\"Chaser: Running Phase 3 Sub-Phase 4\""
  String Constant1 : StringConstant  String="\"Target: Running Phase 3 Sub-Phase 4\""
  String Constant2 : StringConstant  String="\"Obstacle: Running Phase 3 Sub-Phase 4\""
  wires:
  Desired Position BLUE/1(Target Array) -> Data Store Write18/1
  Desired Position RED/1(Target Array) -> Data Store Write9/1
  Desired Joint Angles RED/1(Target Array) -> Data Store Write13/1
  Constant12/1 -> Data Store Write1/1
  Constant18/1 -> Data Store Write2/1
  Constant6/1 -> Data Store Write7/1
  Constant15/1 -> Data Store Write22/1
  Constant14/1 -> Data Store Write23/1
  Constant5/1 -> Data Store Write3/1
  Constant11/1 -> Data Store Write24/1
  Constant8/1 -> Data Store Write16/1
  Constant4/1 -> Data Store Write4/1
  String Constant2/1 -> Data Store Write11/1
  String Constant1/1 -> Data Store Write10/1
  String Constant/1 -> Data Store Write6/1
  Desired Position BLACK/1(Target Array) -> Data Store Write5/1

== system Template_v5_0_0_2026a_Original/1 - Experiment Logic/Phase #4: Return Home/Desired Joint Angles RED ==
  Constant1 : Constant  Value=pi/2
  Constant2 : Constant  Value=0
  Constant3 : Constant  Value=pi/2
  Mux : Mux  Inputs=3
  Target Array : Outport
  wires:
  Mux/1 -> Target Array/1
  Constant3/1 -> Mux/1
  Constant1/1 -> Mux/2
  Constant2/1 -> Mux/3

== system Template_v5_0_0_2026a_Original/1 - Experiment Logic/Phase #4: Return Home/Desired Position BLACK ==
  Desired States (BLACK) : Constant  Value=home_states_BLACK  SampleTime=-1
  Target Array : Outport
  wires:
  Desired States (BLACK)/1 -> Target Array/1

== system Template_v5_0_0_2026a_Original/1 - Experiment Logic/Phase #4: Return Home/Desired Position BLUE ==
  Desired States (BLUE) : Constant  Value=home_states_BLUE  SampleTime=-1
  Target Array : Outport
  wires:
  Desired States (BLUE)/1 -> Target Array/1

== system Template_v5_0_0_2026a_Original/1 - Experiment Logic/Phase #4: Return Home/Desired Position RED ==
  Constant2 : Constant  Value=home_states_RED
  Target Array : Outport
  wires:
  Constant2/1 -> Target Array/1

== system Template_v5_0_0_2026a_Original/1 - Experiment Logic/Phase #5: Hold Home/Desired Joint Angles RED ==
  Constant1 : Constant  Value=pi/2
  Constant2 : Constant  Value=0
  Constant3 : Constant  Value=pi/2
  Mux : Mux  Inputs=3
  Target Array : Outport
  wires:
  Mux/1 -> Target Array/1
  Constant3/1 -> Mux/1
  Constant1/1 -> Mux/2
  Constant2/1 -> Mux/3

== system Template_v5_0_0_2026a_Original/1 - Experiment Logic/Phase #5: Hold Home/Desired Position BLACK ==
  Desired States (BLACK) : Constant  Value=home_states_BLACK  SampleTime=-1
  Target Array : Outport
  wires:
  Desired States (BLACK)/1 -> Target Array/1

== system Template_v5_0_0_2026a_Original/1 - Experiment Logic/Phase #5: Hold Home/Desired Position BLUE ==
  Desired States (BLUE) : Constant  Value=home_states_BLUE  SampleTime=-1
  Target Array : Outport
  wires:
  Desired States (BLUE)/1 -> Target Array/1

== system Template_v5_0_0_2026a_Original/1 - Experiment Logic/Phase #5: Hold Home/Desired Position RED ==
  Constant2 : Constant  Value=home_states_RED
  Target Array : Outport
  wires:
  Constant2/1 -> Target Array/1

== system Template_v5_0_0_2026a_Original/3 - Guidance/Custom PPL (ARM)/Desired Position ==
  Data Store Read : DataStoreRead  DataStoreName=ARM_Desired_States  IndexOptions=Index vector (dialog)  Indices=1  OutputSizes=1
  Position Array : Outport
  wires:
  Data Store Read/1 -> Position Array/1

== system Template_v5_0_0_2026a_Original/3 - Guidance/Custom PPL (BLACK)/Desired Position ==
  BLACK_Px : DataStoreRead  DataStoreName=BLACK_Desired_States  IndexOptions=Index vector (dialog)  Indices=1  OutputSizes=1
  Position Array : Outport
  wires:
  BLACK_Px/1 -> Position Array/1

== system Template_v5_0_0_2026a_Original/3 - Guidance/Custom PPL (BLUE)/Desired Position ==
  Data Store Read4 : DataStoreRead  DataStoreName=BLUE_Desired_States  IndexOptions=Index vector (dialog)  Indices=1  OutputSizes=1
  Position Array : Outport
  wires:
  Data Store Read4/1 -> Position Array/1

== system Template_v5_0_0_2026a_Original/3 - Guidance/Custom PPL (RED)/Desired Position ==
  RED_Px : DataStoreRead  DataStoreName=RED_Desired_States  IndexOptions=Index vector (dialog)  Indices=1  OutputSizes=1
  Position Array : Outport
  wires:
  RED_Px/1 -> Position Array/1

== system Template_v5_0_0_2026a_Original/3 - Guidance/Disable PPL (ARM)/Desired Position ==
  Data Store Read : DataStoreRead  DataStoreName=ARM_Desired_States  IndexOptions=Index vector (dialog)  Indices=1  OutputSizes=1
  Position Array : Outport
  wires:
  Data Store Read/1 -> Position Array/1

== system Template_v5_0_0_2026a_Original/3 - Guidance/Disable PPL (BLACK)/Desired Position ==
  BLACK_Px : DataStoreRead  DataStoreName=BLACK_Desired_States  IndexOptions=Index vector (dialog)  Indices=1  OutputSizes=1
  Position Array : Outport
  wires:
  BLACK_Px/1 -> Position Array/1

== system Template_v5_0_0_2026a_Original/3 - Guidance/Disable PPL (BLUE)/Desired Position ==
  Data Store Read4 : DataStoreRead  DataStoreName=BLUE_Desired_States  IndexOptions=Index vector (dialog)  Indices=1  OutputSizes=1
  Position Array : Outport
  wires:
  Data Store Read4/1 -> Position Array/1

== system Template_v5_0_0_2026a_Original/3 - Guidance/Disable PPL (RED)/Desired Position ==
  RED_Px : DataStoreRead  DataStoreName=RED_Desired_States  IndexOptions=Index vector (dialog)  Indices=1  OutputSizes=1
  Position Array : Outport
  wires:
  RED_Px/1 -> Position Array/1

== system Template_v5_0_0_2026a_Original/4 - Control/Default LQR Control (BLACK)/Calculate Error ==
  Desired Attitude : Inport
  Measured Attitude : Inport  Port=2
  MATLAB Function : MATLAB Function  TreatAsAtomicUnit=on
  Attitude Error : Outport
  wires:
  MATLAB Function/1(Rz_error) -> Attitude Error/1
  Desired Attitude/1 -> MATLAB Function/1(Rz_path)
  Measured Attitude/1 -> MATLAB Function/2(Rz_measured)

== system Template_v5_0_0_2026a_Original/4 - Control/Default LQR Control (BLUE)/Calculate Error ==
  Desired Attitude : Inport
  Measured Attitude : Inport  Port=2
  MATLAB Function : MATLAB Function  TreatAsAtomicUnit=on
  Attitude Error : Outport
  wires:
  MATLAB Function/1(Rz_error) -> Attitude Error/1
  Desired Attitude/1 -> MATLAB Function/1(Rz_path)
  Measured Attitude/1 -> MATLAB Function/2(Rz_measured)

== system Template_v5_0_0_2026a_Original/4 - Control/Default LQR Control (RED)/Calculate Error ==
  Desired Attitude : Inport
  Measured Attitude : Inport  Port=2
  MATLAB Function : MATLAB Function  TreatAsAtomicUnit=on
  Attitude Error : Outport
  wires:
  MATLAB Function/1(Rz_error) -> Attitude Error/1
  Desired Attitude/1 -> MATLAB Function/1(Rz_path)
  Measured Attitude/1 -> MATLAB Function/2(Rz_measured)

== system Template_v5_0_0_2026a_Original/PhaseSpace Camera Code/Use Hardware to Obtain States/Receive and Process Phasespace Data ==
  Demux2 : Demux  Outputs=[1,18,96]
  Experiment Clock : Subsystem
  LED Terminator : Terminator
  Mux : Mux  Inputs=2
  Receive PhaseSpace Data : MATLAB Function  TreatAsAtomicUnit=on
  Reshape : Reshape  OutputDimensionality=Customize  OutputDimensions=[115,1]
  Terminator : Terminator
  To double : DataTypeConversion  OutDataTypeStr=double  SaturateOnIntegerOverflow=off  RndMeth=Floor
  PhaseSpace Data : Outport
  PhaseSpace Clock : Outport  Port=2
  wires:
  Reshape/1 -> Demux2/1
  Demux2/2 -> Mux/2
  Mux/1 -> PhaseSpace Data/1
  Demux2/1 -> PhaseSpace Clock/1
  Experiment Clock/1(ClockAdjusted) -> Mux/1
  Receive PhaseSpace Data/1(packet) -> To double/1, Experiment Clock/1(packet)
  To double/1 -> Reshape/1
  Demux2/3 -> LED Terminator/1
  Receive PhaseSpace Data/2(newPackets) -> Terminator/1
  Receive PhaseSpace Data/3(age) -> Experiment Clock/2(age)

== system Template_v5_0_0_2026a_Original/PhaseSpace Camera Code/Use Hardware to Obtain States/Store BLACK Data ==
  note: Store BLACK Positions and Velocities
  BLACK Data : Inport
  BLACK Velocities : Inport  Port=2
  PS Clock : Inport  Port=3
  Calculate True Time Step : Subsystem
      settings: PortSchema="{\"entries\":[{\"content\":{\"sides\":[{\"content\":{\"connectorIds\":[\"In1\"]},\"type\":\"ConnectorPlacement.EquallySpacedRectSide\",\"uuid\":\"62932c5c-f2a7-44c8-96b4-4a75bab3a126\"},{\"content\":{\"connectorIds\":[\"Out1\"],\"side\":\"RIGHT\"},\"type\":\"ConnectorPlacement.EquallySpacedRectSide\",\"uuid\":\"82b3b717-2171-4047-b0df-3cd41cf9dfc7\"},{\"content\":{\"side\":\"TOP\"},\"type\":\"ConnectorPlacement.EquallySpacedRectSide\",\"uuid\":\"a142272a-a0ff-4882-8a2d-4633b3c7e02f\"},{\"content\":{\"connectorIds\":[\"In2\"],\"side\":\"BOTTOM\"},\"type\":\"ConnectorPlacement.EquallySpacedRectSide\",\"uuid\":\"b1e1ff4c-66d6-488f-92fb-77f76780833b\"}]},\"type\":\"ConnectorPlacement.EquallySpacedConnector\",\"uuid\":\"98c51868-8a10-4b52-aae4-56f6042c65c4\"}],\"packageUris\":[\"http://schema.mathworks.com/mf0/Connector/R2020b\"],\"version\":\"1.0\"}"
  Convert BLACKVX from [mm] to [m] : Gain  Gain=1/1000
  Convert BLACKVY from [mm] to [m] : Gain  Gain=1/1000
  Convert BLAX from [mm] to [m] : Gain  Gain=1/1000
  Convert BLAY from [mm] to [m] : Gain  Gain=1/1000
  Demux : Demux  Outputs=3
  Demux2 : Demux  Outputs=3
  Demux3 : Demux  Outputs=3
  Mux{1..4} (4 alike) : Mux  Inputs=3
  RED_Px7 : DataStoreWrite  DataStoreName=BLACK_Measured_States  IndexOptions=Index vector (dialog)  Indices=1  OutputSizes=1
  Reshape : Reshape  OutputDimensionality=Column vector (2-D)
  Subsystem1 : Subsystem
  Subsystem2 : Subsystem
  Wrap : Subsystem
  wires:
  Demux3/1 -> Convert BLAX from [mm] to [m]/1
  Demux3/2 -> Convert BLAY from [mm] to [m]/1
  BLACK Data/1 -> Demux3/1
  Demux/3 -> Wrap/1(Unwrapped Angle)
  Reshape/1 -> Subsystem1/2(y)
  Demux/1 -> Mux1/1
  Convert BLAY from [mm] to [m]/1 -> Mux3/2
  Calculate True Time Step/1(dt_out) -> Subsystem2/1(dt), Subsystem1/1(dt)
  Mux3/1 -> Subsystem2/2(y), Demux/1, Calculate True Time Step/2(Data)
  Wrap/1(Wrapped Angle) -> Mux1/3
  Convert BLAX from [mm] to [m]/1 -> Mux3/1
  Mux2/1 -> RED_Px7/1
  Demux/2 -> Mux1/2
  Subsystem2/1(dy/dt) -> Reshape/1
  PS Clock/1 -> Calculate True Time Step/1(Time)
  Demux3/3 -> Mux3/3
  Mux1/1 -> Mux2/1
  Subsystem1/1(dy/dt) -> Mux2/3
  BLACK Velocities/1 -> Demux2/1
  Demux2/3 -> Mux4/3
  Convert BLACKVX from [mm] to [m]/1 -> Mux4/1
  Convert BLACKVY from [mm] to [m]/1 -> Mux4/2
  Mux4/1 -> Mux2/2
  Demux2/2 -> Convert BLACKVY from [mm] to [m]/1
  Demux2/1 -> Convert BLACKVX from [mm] to [m]/1

== system Template_v5_0_0_2026a_Original/PhaseSpace Camera Code/Use Hardware to Obtain States/Store BLUE Data ==
  note: Store BLUE Positions and Velocities
  BLUE Data : Inport
  BLUE Velocities : Inport  Port=2
  PS Clock : Inport  Port=3
  Calculate True Time Step : Subsystem
      settings: PortSchema="{\"entries\":[{\"content\":{\"sides\":[{\"content\":{\"connectorIds\":[\"In1\"]},\"type\":\"ConnectorPlacement.EquallySpacedRectSide\",\"uuid\":\"62932c5c-f2a7-44c8-96b4-4a75bab3a126\"},{\"content\":{\"connectorIds\":[\"Out1\"],\"side\":\"RIGHT\"},\"type\":\"ConnectorPlacement.EquallySpacedRectSide\",\"uuid\":\"82b3b717-2171-4047-b0df-3cd41cf9dfc7\"},{\"content\":{\"side\":\"TOP\"},\"type\":\"ConnectorPlacement.EquallySpacedRectSide\",\"uuid\":\"a142272a-a0ff-4882-8a2d-4633b3c7e02f\"},{\"content\":{\"connectorIds\":[\"In2\"],\"side\":\"BOTTOM\"},\"type\":\"ConnectorPlacement.EquallySpacedRectSide\",\"uuid\":\"b1e1ff4c-66d6-488f-92fb-77f76780833b\"}]},\"type\":\"ConnectorPlacement.EquallySpacedConnector\",\"uuid\":\"98c51868-8a10-4b52-aae4-56f6042c65c4\"}],\"packageUris\":[\"http://schema.mathworks.com/mf0/Connector/R2020b\"],\"version\":\"1.0\"}"
  Convert BLUEVX from [mm] to [m] : Gain  Gain=1/1000
  Convert BLUEVY from [mm] to [m] : Gain  Gain=1/1000
  Convert BLUX from [mm] to [m] : Gain  Gain=1/1000
  Convert BLUY from [mm] to [m] : Gain  Gain=1/1000
  Demux : Demux  Outputs=3
  Demux2 : Demux  Outputs=3
  Demux5 : Demux  Outputs=3
  Mux{1..4} (4 alike) : Mux  Inputs=3
  RED_Px7 : DataStoreWrite  DataStoreName=BLUE_Measured_States  IndexOptions=Index vector (dialog)  Indices=1  OutputSizes=1
  Reshape : Reshape  OutputDimensionality=Column vector (2-D)
  Subsystem1 : Subsystem
  Subsystem2 : Subsystem
  Wrap : Subsystem
  wires:
  Demux5/2 -> Convert BLUY from [mm] to [m]/1
  Demux5/1 -> Convert BLUX from [mm] to [m]/1
  BLUE Data/1 -> Demux5/1
  Calculate True Time Step/1(dt_out) -> Subsystem2/1(dt), Subsystem1/1(dt)
  Demux/2 -> Mux1/2
  Demux/1 -> Mux1/1
  Subsystem2/1(dy/dt) -> Reshape/1
  Mux3/1 -> Subsystem2/2(y), Demux/1, Calculate True Time Step/2(Data)
  Demux/3 -> Wrap/1(Unwrapped Angle)
  Reshape/1 -> Subsystem1/2(y)
  Wrap/1(Wrapped Angle) -> Mux1/3
  Mux2/1 -> RED_Px7/1
  Convert BLUY from [mm] to [m]/1 -> Mux3/2
  Convert BLUX from [mm] to [m]/1 -> Mux3/1
  Demux5/3 -> Mux3/3
  PS Clock/1 -> Calculate True Time Step/1(Time)
  Mux1/1 -> Mux2/1
  Subsystem1/1(dy/dt) -> Mux2/3
  Demux2/1 -> Convert BLUEVX from [mm] to [m]/1
  Convert BLUEVY from [mm] to [m]/1 -> Mux4/2
  BLUE Velocities/1 -> Demux2/1
  Demux2/2 -> Convert BLUEVY from [mm] to [m]/1
  Mux4/1 -> Mux2/2
  Demux2/3 -> Mux4/3
  Convert BLUEVX from [mm] to [m]/1 -> Mux4/1
